simulink model "geometric_control_template"  (R2024b)
settings: Solver=VariableStepAuto  StartTime=0.0  StopTime=30.0  RelTol=1e-3
InitFcn:
  | %% INITIALIZATION
  | 
  | %% UAV PARAMETERS
  | 
  | mass = 1.2;
  | Ib = diag([1.2416 1.2416 2*1.2416]);
  | 
  | %% SAMPLING TIME
  | Ts=0.001;
  | 
  | %% PLANNER
  | t_iniz = 0;
  | ttot=20; %duration
  | tdead=10; %dead time to evaluate the steady-state
  | tot_time = ttot + tdead;
  | t1=linspace(0,ttot,round(ttot/Ts));
  | t=linspace(0,ttot+tdead,round(ttot/Ts)+round(tdead/Ts));
  | p= zeros(4,length(t1)); dot_p= zeros(4,length(t1)); ddot_p= zeros(4,length(t1));
  | p_d= zeros(4,length(t)); dot_p_d= zeros(4,length(t)); ddot_p_d= zeros(4,length(t));
  | %Initial and final conditions
  | x0= 0; xf=1; dot_x0= 0; dot_xf=0; ddot_x0=0; ddot_xf=0; dddot_x0 = 0; dddot_xf = 0;
  | y0= 0; yf=1; dot_y0= 0; dot_yf=0; ddot_y0=0; ddot_yf=0; dddot_y0 = 0; dddot_yf = 0;
  | z0= -1; zf=-4; dot_z0= 0; dot_zf=0; ddot_z0=0; ddot_zf=0; dddot_z0 = 0; dddot_zf = 0;
  | psi0 = 0;
  | psif=deg2rad(20); dot_psi0= 0; dot_psif=0; ddot_psi0=0; ddot_psif=0; dddot_psi0 = 0; dddot_psif = 0;
  | p0=[x0,y0,z0,psi0]; dot_p0=[dot_x0,dot_y0,dot_z0,dot_psi0]; ddot_p0=[ddot_x0,ddot_y0,ddot_z0,ddot_psi0]; dddot_p0=[dddot_x0,dddot_y0,dddot_z0,dddot_psi0];
  | pf=[xf,yf,zf,psif]; dot_pf=[dot_xf,dot_yf,dot_zf,dot_psif]; ddot_pf=[ddot_xf,ddot_yf,ddot_zf,ddot_psif]; dddot_pf=[dddot_xf,dddot_yf,dddot_zf,dddot_psif];
  | %5-th order polynomial
  | a0=zeros(1,4); a1=zeros(1,4); a2=zeros(1,4); a3=zeros(1,4); a4=zeros(1,4); a5=zeros(1,4); a6 = zeros(1,4); a7 = zeros(1,4);
  | 
  | for j=1:4
  |     A = [t_iniz^7, t_iniz^6, t_iniz^5, t_iniz^4, t_iniz^3, t_iniz^2, t_iniz, 1;
  |         ttot^7, ttot^6, ttot^5, ttot^4, ttot^3, ttot^2, ttot, 1;
  |         7*t_iniz^6, 6*t_iniz^5, 5*t_iniz^4, 4*t_iniz^3, 3*t_iniz^2, 2*t_iniz, 1, 0;
  |         7*ttot^6, 6*ttot^5, 5*ttot^4, 4*ttot^3, 3*ttot^2, 2*ttot, 1, 0;
  |         42*t_iniz^5, 30*t_iniz^4, 20*t_iniz^3, 12*t_iniz^2, 6*t_iniz, 2, 0, 0;
  |         42*ttot^5, 30*ttot^4, 20*ttot^3, 12*ttot^2, 6*ttot, 2, 0, 0;
  |         210*t_iniz^4, 120*t_iniz^3, 60*t_iniz^2, 24*t_iniz, 6, 0, 0, 0;
  |         210*ttot^4, 120*ttot^3, 60*ttot^2, 24*ttot, 6, 0, 0, 0];
  |     b = [p0(j) pf(j) dot_p0(j) dot_pf(j) ddot_p0(j) ddot_pf(j) dddot_p0(j) dddot_pf(j)]';
  |     a_temp = A\b;
  |     a7(j) = a_temp(1);
  |     a6(j) = a_temp(2);
  |     a5(j) = a_temp(3);
  |     a4(j) = a_temp(4);
  |     a3(j) = a_temp(5);
  |     a2(j) = a_temp(6);
  |     a1(j) = a_temp(7);
  |     a0(j) = a_temp(8);
  | 
  |     %trajectories
  |     p(j,:)=a7(j)*t1.^7 + a6(j)*t1.^6 + a5(j)*t1.^5 +a4(j)*t1.^4 +a3(j)*t1.^3 +a2(j)*t1.^2 +a1(j)*t1 +a0(j);
  |     dot_p(j,:) = 7*a7(j)*t1.^6 + 6*a6(j)*t1.^5 + 5*a5(j)*t1.^4 +4*a4(j)*t1.^3 +3*a3(j)*t1.^2 +2*a2(j)*t1 +a1(j);
  |     ddot_p(j,:) = 42*a7(j)*t1.^5 + 30*a6(j)*t1.^4 + 5*4*a5(j)*t1.^3 +4*3*a4(j)*t1.^2 +3*2*a3(j)*t1 +2*a2(j);
  |     %addition of the stead-state terms
  |     p_d(j,:)=[p(j,:) zeros(1,round(tdead/Ts))+pf(j)];
  |     dot_p_d(j,:)=[dot_p(j,:) zeros(1,round(tdead/Ts))+dot_pf(j)];
  |     ddot_p_d(j,:)=[ddot_p(j,:) zeros(1,round(tdead/Ts))+ddot_pf(j)];
  | end
  | %data for Simulink
  | pos_0 = [x0 y0 z0];
  | lin_vel_0 = [dot_x0 dot_y0 dot_z0];
  | w_bb_0 = [0 0 0];
  | csi_d=p_d(1:3,:); dot_csi_d=dot_p_d(1:3,:); ddot_csi_d=ddot_p_d(1:3,:);
  | psi_d=p_d(4,:); dot_psi_d=dot_p_d(4,:); ddot_psi_d=ddot_p_d(4,:);
libraries: robotcorelib x1, uavutilslib x1
settings Model: Creator=fabioruggiero  LastModifiedBy=feder
settings ModelReferenceCC: EnableRefExpFcnMdlSchedulingChecks=on
settings RTWCC: GPUComputeCapability=3.5

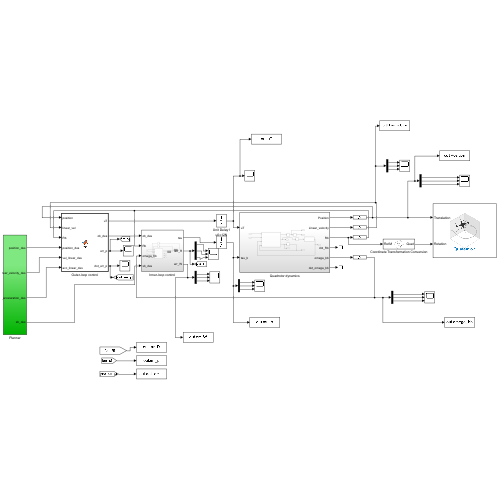
[thumbnail: Simulink's stored preview of the top-level diagram]
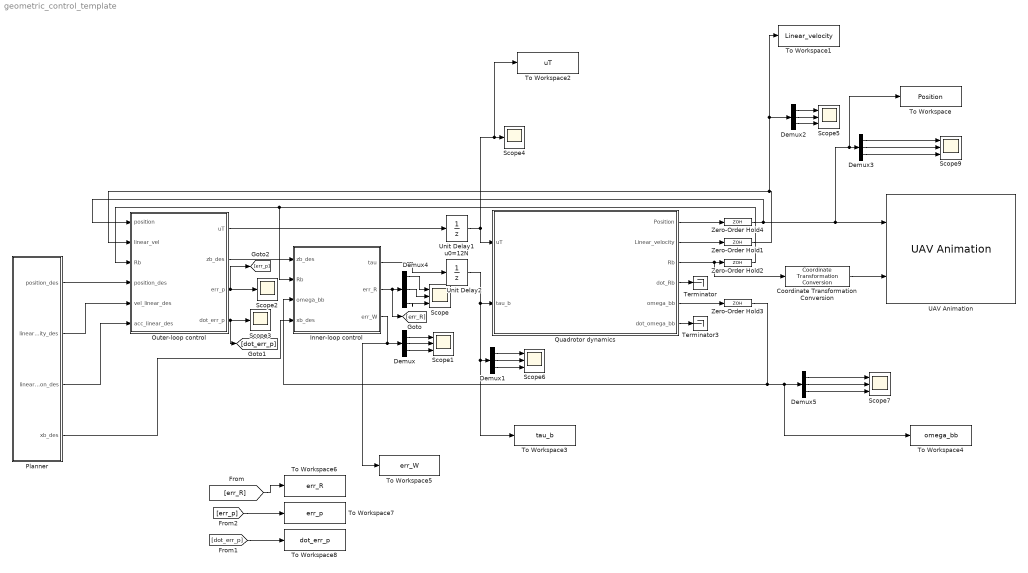
== system geometric_control_template ==
  Coordinate Transformation Conversion : robotcorelib/Coordinate Transformation Conversion  InputRepresentation=Rotation Matrix  InputEulerSequence=ZYX  ShowTrVecInputPort=on  OutputRepresentation=Quaternion  OutputEulerSequence=ZYX  ShowTrVecOutputPort=on  SimulateUsing=Interpreted execution
  Demux{,1..5} (6 alike) : Demux  Outputs=3
  Inner-loop control : Subsystem
  Outer-loop control : MATLAB Function  TreatAsAtomicUnit=on
  Planner : Subsystem
  Quadrotor dynamics : Subsystem
  Scope{,1,5..7,9} (6 alike) : Scope  NumInputPorts=3
  Scope2 : Scope
  Scope3 : Scope
  Scope4 : Scope
  Terminator : Terminator
  Terminator3 : Terminator
  To Workspace : ToWorkspace  VariableName=Position  SaveFormat=Timeseries  SampleTime=-1
  To Workspace1 : ToWorkspace  VariableName=Linear_velocity  SaveFormat=Timeseries  SampleTime=-1
  To Workspace2 : ToWorkspace  VariableName=uT  SaveFormat=Timeseries  SampleTime=-1
  To Workspace3 : ToWorkspace  VariableName=tau_b  SaveFormat=Timeseries  SampleTime=-1
  To Workspace4 : ToWorkspace  VariableName=omega_bb  SaveFormat=Timeseries  SampleTime=-1
  To Workspace5 : ToWorkspace  VariableName=err_W  SaveFormat=Timeseries  SampleTime=-1
  To Workspace6 : ToWorkspace  VariableName=err_R  SaveFormat=Timeseries  SampleTime=-1
  To Workspace7 : ToWorkspace  VariableName=err_p  SaveFormat=Timeseries  SampleTime=-1
  To Workspace8 : ToWorkspace  VariableName=dot_err_p  SaveFormat=Timeseries  SampleTime=-1
  UAV Animation : uavutilslib/UAV Animation  NumUAV=1  DynamicUAVConfig=off  UAVType=Multirotor  UAVSize=1  UAVColor=[1 0 0]  UAVTrajectoryAlpha=1  InertialZDirection=Down  RotationFormat=Quaternion  DrawMarkers=off  SampleTime=0.01
  Unit Delay1 u0=12N : UnitDelay  InitialCondition=12  SampleTime=Ts
  Unit Delay2 : UnitDelay  InitialCondition=[0 0 0]  SampleTime=Ts
  Zero-Order Hold{1..4} (4 alike) : ZeroOrderHold  SampleTime=Ts
  wires:
  Outer-loop control/1(uT) -> Unit Delay1 u0=12N/1
  Unit Delay1 u0=12N/1 -> Quadrotor dynamics/1(uT), To Workspace2/1, Scope4/1
  Quadrotor dynamics/1(Position) -> Zero-Order Hold4/1
  Quadrotor dynamics/2(Linear_velocity) -> Zero-Order Hold1/1
  Quadrotor dynamics/3(Rb) -> Coordinate Transformation Conversion/1, Zero-Order Hold2/1
  Quadrotor dynamics/5(omega_bb) -> Zero-Order Hold3/1
  Zero-Order Hold4/1 -> To Workspace/1, Demux3/1, UAV Animation/1, Outer-loop control/1(position)
  Zero-Order Hold1/1 -> Demux2/1, To Workspace1/1, Outer-loop control/2(linear_vel)
  Zero-Order Hold2/1 -> Outer-loop control/3(Rb), Inner-loop control/2(Rb)
  Unit Delay2/1 -> To Workspace3/1, Demux1/1, Quadrotor dynamics/2(tau_b)
  Quadrotor dynamics/4(dot_Rb) -> Terminator/1
  Planner/1(position_des) -> Outer-loop control/4(position_des)
  Planner/2(linear_velocity_des) -> Outer-loop control/5(vel_linear_des)
  Planner/3(linear_acceleration_des) -> Outer-loop control/6(acc_linear_des)
  Planner/4(xb_des) -> Inner-loop control/4(xb_des)
  Outer-loop control/3(err_p) -> Scope2/1, [err_p]
  Outer-loop control/4(dot_err_p) -> [dot_err_p], Scope3/1
  Quadrotor dynamics/6(dot_omega_bb) -> Terminator3/1
  Coordinate Transformation Conversion/1 -> UAV Animation/2
  Outer-loop control/2(zb_des) -> Inner-loop control/1(zb_des)
  Zero-Order Hold3/1 -> To Workspace4/1, Demux5/1, Inner-loop control/3(omega_bb)
  Inner-loop control/1(tau) -> Unit Delay2/1
  Demux3/1 -> Scope9/1
  Demux3/3 -> Scope9/3
  Demux3/2 -> Scope9/2
  Demux1/1 -> Scope6/1
  Demux1/3 -> Scope6/3
  Demux1/2 -> Scope6/2
  Demux2/2 -> Scope5/2
  Demux2/3 -> Scope5/3
  Demux2/1 -> Scope5/1
  Demux5/1 -> Scope7/1
  Demux5/2 -> Scope7/2
  Demux5/3 -> Scope7/3
  Inner-loop control/3(err_W) -> Demux/1, To Workspace5/1
  Demux/1 -> Scope1/1
  Demux/2 -> Scope1/2
  Demux/3 -> Scope1/3
  Inner-loop control/2(err_R) -> Demux4/1, [err_R]
  Demux4/1 -> Scope/1
  Demux4/2 -> Scope/2
  Demux4/3 -> Scope/3
  [err_R] -> To Workspace6/1
  [dot_err_p] -> To Workspace8/1
  [err_p] -> To Workspace7/1

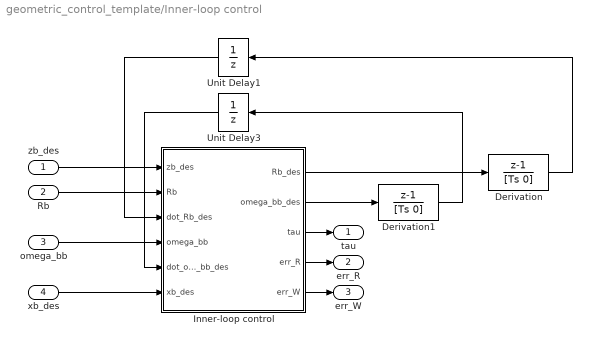
== system geometric_control_template/Inner-loop control ==
  zb_des : Inport
  Rb : Inport  Port=2
  omega_bb : Inport  Port=3
  xb_des : Inport  Port=4
  Derivation : DiscreteTransferFcn  Numerator=[1 -1]  Denominator=[Ts 0]  InitialStates=[1 0 0;0 1 0;0 0 1]  SampleTime=Ts
  Derivation1 : DiscreteTransferFcn  Numerator=[1 -1]  Denominator=[Ts 0]  InitialStates=[0 0 0]  SampleTime=Ts
  Inner-loop control : MATLAB Function  TreatAsAtomicUnit=on
  Unit Delay1 : UnitDelay  InitialCondition=eye(3)  SampleTime=Ts
  Unit Delay3 : UnitDelay  InitialCondition=[0 0 0]  SampleTime=Ts
  tau : Outport
  err_R : Outport  Port=2
  err_W : Outport  Port=3
  wires:
  xb_des/1 -> Inner-loop control/6(xb_des)
  Inner-loop control/4(err_R) -> err_R/1
  Rb/1 -> Inner-loop control/2(Rb)
  Inner-loop control/3(tau) -> tau/1
  Unit Delay1/1 -> Inner-loop control/3(dot_Rb_des)
  Derivation1/1 -> Unit Delay3/1
  Inner-loop control/5(err_W) -> err_W/1
  Unit Delay3/1 -> Inner-loop control/5(dot_omega_bb_des)
  Derivation/1 -> Unit Delay1/1
  zb_des/1 -> Inner-loop control/1(zb_des)
  omega_bb/1 -> Inner-loop control/4(omega_bb)
  Inner-loop control/1(Rb_des) -> Derivation/1
  Inner-loop control/2(omega_bb_des) -> Derivation1/1

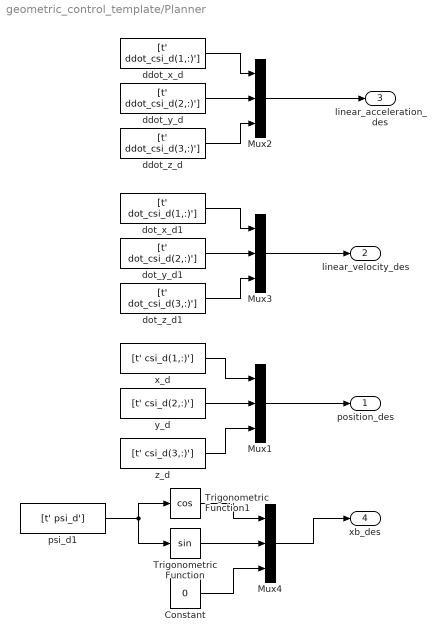
== system geometric_control_template/Planner ==
  Constant : Constant  Value=0
  Mux{1..4} (4 alike) : Mux  Inputs=3
  Trigonometric Function : Trigonometry
  Trigonometric Function1 : Trigonometry  Operator=cos
  ddot_x_d : FromWorkspace  VariableName=[t' ddot_csi_d(1,:)']  SampleTime=Ts
  ddot_y_d : FromWorkspace  VariableName=[t' ddot_csi_d(2,:)']  SampleTime=Ts
  ddot_z_d : FromWorkspace  VariableName=[t' ddot_csi_d(3,:)']  SampleTime=Ts
  dot_x_d1 : FromWorkspace  VariableName=[t' dot_csi_d(1,:)']  SampleTime=Ts
  dot_y_d1 : FromWorkspace  VariableName=[t' dot_csi_d(2,:)']  SampleTime=Ts
  dot_z_d1 : FromWorkspace  VariableName=[t' dot_csi_d(3,:)']  SampleTime=Ts
  psi_d1 : FromWorkspace  VariableName=[t' psi_d']  SampleTime=Ts
  x_d : FromWorkspace  VariableName=[t' csi_d(1,:)']  SampleTime=Ts
  y_d : FromWorkspace  VariableName=[t' csi_d(2,:)']  SampleTime=Ts
  z_d : FromWorkspace  VariableName=[t' csi_d(3,:)']  SampleTime=Ts
  position_des : Outport
  linear_velocity_des : Outport  Port=2
  linear_acceleration_des : Outport  Port=3
  xb_des : Outport  Port=4
  wires:
  y_d/1 -> Mux1/2
  z_d/1 -> Mux1/3
  x_d/1 -> Mux1/1
  ddot_y_d/1 -> Mux2/2
  ddot_z_d/1 -> Mux2/3
  ddot_x_d/1 -> Mux2/1
  Mux2/1 -> linear_acceleration_des/1
  Mux1/1 -> position_des/1
  dot_y_d1/1 -> Mux3/2
  dot_z_d1/1 -> Mux3/3
  dot_x_d1/1 -> Mux3/1
  Mux3/1 -> linear_velocity_des/1
  Mux4/1 -> xb_des/1
  Trigonometric Function/1 -> Mux4/2
  psi_d1/1 -> Trigonometric Function/1, Trigonometric Function1/1
  Trigonometric Function1/1 -> Mux4/1
  Constant/1 -> Mux4/3

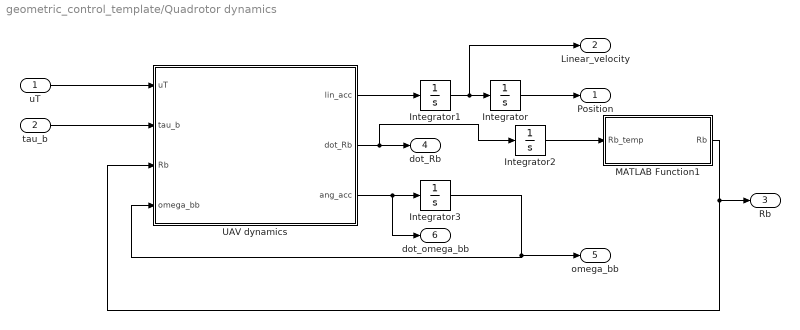
== system geometric_control_template/Quadrotor dynamics ==
  uT : Inport
  tau_b : Inport  Port=2
  Integrator : Integrator  InitialCondition=pos_0
  Integrator1 : Integrator  InitialCondition=lin_vel_0
  Integrator2 : Integrator  InitialCondition=[1 0 0; 0 1 0;0 0 1]
  Integrator3 : Integrator  InitialCondition=w_bb_0
  MATLAB Function1 : MATLAB Function  TreatAsAtomicUnit=on
  UAV dynamics : MATLAB Function  TreatAsAtomicUnit=on
  Position : Outport
  Linear_velocity : Outport  Port=2
  Rb : Outport  Port=3
  dot_Rb : Outport  Port=4
  omega_bb : Outport  Port=5
  dot_omega_bb : Outport  Port=6
  wires:
  tau_b/1 -> UAV dynamics/2(tau_b)
  Integrator/1 -> Position/1
  UAV dynamics/3(ang_acc) -> dot_omega_bb/1, Integrator3/1
  UAV dynamics/1(lin_acc) -> Integrator1/1
  uT/1 -> UAV dynamics/1(uT)
  Integrator1/1 -> Linear_velocity/1, Integrator/1
  Integrator3/1 -> UAV dynamics/4(omega_bb), omega_bb/1
  UAV dynamics/2(dot_Rb) -> Integrator2/1, dot_Rb/1
  MATLAB Function1/1(Rb) -> Rb/1, UAV dynamics/3(Rb)
  Integrator2/1 -> MATLAB Function1/1(Rb_temp)

== matlab function geometric_control_template/Quadrotor dynamics/UAV dynamics ==
  data: uT input size=1; tau_b input size=3; lin_acc output size=3; Rb input size=[3,3]; omega_bb input size=3; dot_Rb output size=[3,3]; ang_acc output size=3; mass parameter size=1; Ib parameter size=[3,3]
function [lin_acc, dot_Rb, ang_acc] = fcn(uT,tau_b,Rb,omega_bb,mass, Ib)

lin_acc = 9.81*[0 0 1]'-(uT/mass)*Rb*[0 0 1]';
dot_Rb = Rb*skew(omega_bb);
ang_acc = inv(Ib)*(-skew(omega_bb)*Ib*omega_bb + tau_b);

end

function S = skew(v)
if(numel(v)~= 1)
S= [0 -v(3) v(2); 
    v(3) 0 -v(1);
    -v(2) v(1) 0];
else
S= zeros(3);
end
end

== matlab function geometric_control_template/Outer-loop control ==
  data: position input size=3; uT output size=1; linear_vel input size=3; Rb input size=[3,3]; zb_des output size=3; mass parameter size=1; position_des input size=3; vel_linear_des input size=3; acc_linear_des input size=3; err_p output size=3; dot_err_p output size=3
function [uT, zb_des, err_p, dot_err_p] = fcn(position, linear_vel, Rb, mass, ...
    position_des, vel_linear_des, acc_linear_des)

%% WRITE HERE THE OUTER-LOOP CONTROL
% position: linear position measure
% linear_vel: linear velocity measure
% Rb: current rotation matrix
% mass: mass of the UAV
% positon_des: desired linear position from the planner
% vel_linear_des: desired linear velocity from the planner
% acc_linear_des: desired linear acceleration from the planner
% ---
% uT: commanded total thrust
% zb_des: desired z-axis of the body frame
% err_p: position error
% dot_err_p: time derivative of the positon error


K_p=10*eye(3);
K_v=10*eye(3);

g=9.81;
e3=[0 0 1]';

err_p=position-position_des;
dot_err_p=linear_vel-vel_linear_des;

%slide 71 pdf_4
A = -K_p*err_p-K_v*dot_err_p-mass*g*e3+mass*acc_linear_des; % desired control force for the translational dynamics
uT = -A'*Rb*e3;
zb_des = -A/norm(A);

end

== matlab function geometric_control_template/Inner-loop control/Inner-loop control ==
  data: Rb_des output size=[3,3]; omega_bb_des output size=3; tau output size=3; zb_des input size=3; Rb input size=[3,3]; dot_Rb_des input size=[3,3]; omega_bb input size=3; dot_omega_bb_des input size=3; xb_des input size=3; Ib parameter size=[3,3]; err_R output size=3; err_W output size=3
function [Rb_des,omega_bb_des,tau,err_R,err_W] = fcn(zb_des,Rb,dot_Rb_des,omega_bb,dot_omega_bb_des,xb_des,Ib)

%% WRITE HERE THE INNER-LOOP CONTROL
% zb_des: desired z-axis of the body frame
% Rb: current rotation matrix
% dot_Rb_des: time-derivative of the desired rotation matrix
% omega_bb: current angular velocity expressed in the body frame
% dot_omega_bb_des: desired angular acceleration expressed in the body
% frame
% xb_des: desired x-axis of the body frame form the planner
% Ib: inertia matrix of the UAV with respect to the body frame
% ---
% Rb_des: desired rotation matrix
% omega_bb_des: desired angular velocity expressed in the body frame (given
% below as a hint)
% tau: commanded control torque
% err_R: rotational error in SO(3)
% err_W: angular velocity error in SO(3)


yb_des=skew(zb_des)*xb_des/norm(skew(zb_des)*xb_des); %slide 64
Rb_des=[skew(yb_des)*zb_des, yb_des, zb_des]; 
omega_bb_des = wedge(Rb_des'*dot_Rb_des);
err_R=1/2*wedge((Rb_des'*Rb-Rb'*Rb_des));
err_W=omega_bb-Rb'*Rb_des*omega_bb_des;
K_r=200*eye(3);
K_w=80*eye(3);
tau = -K_r*err_R-K_w*err_W+skew(omega_bb)*Ib*omega_bb-Ib*(skew(omega_bb)*Rb'*Rb_des*omega_bb_des-Rb'*Rb_des*dot_omega_bb_des);

end

function S = skew(v)
if(numel(v)~= 1)
S= [0 -v(3) v(2); 
    v(3) 0 -v(1);
    -v(2) v(1) 0];
else
S= zeros(3);
end
end

function v = wedge(S)
v1 = S(3,2);
v2 = S(1,3);
v3 = S(2,1);
v = [v1 v2 v3]';
end

== matlab function geometric_control_template/Quadrotor dynamics/MATLAB Function1 ==
  data: Rb_temp input; Rb output
function Rb = fcn(Rb_temp)
    [U,S,V] = svd(Rb_temp);
    sigma = det(U*V');
    S_ = diag([1 1 sigma]);

    Rb = U*S_*V';
end
